simulink model "UPS_CRM_PFC"  (R2023b)
settings: Solver=FixedStepAuto  StartTime=0.0  StopTime=0.5  RelTol=1e-3
libraries: spsSeriesRLCBranchLib x7, spsVoltageMeasurementLib x5, spsUniversalBridgeLib x3, spsCurrentMeasurementLib x2, spsACVoltageSourceLib x1, simulink_extras x1, spsMeanLib x1, spsMutualInductanceLib x1, slpidlib x1, powerlib_extras x1, spsTHDLib x1, spspowerguiLib x1
settings Model: SimulationMode=accelerator  Creator=abc6820292  LastModifiedBy=Qu
settings SolverCC: ZeroCrossAlgorithm=Adaptive
settings DebuggingCC: IgnoredZcDiagnostic=none  UnconnectedInputMsg=warning  UnconnectedOutputMsg=warning  UnconnectedLineMsg=warning
settings ModelReferenceCC: EnableRefExpFcnMdlSchedulingChecks=on
settings RTWCC: DLArmComputeVersion=19.05

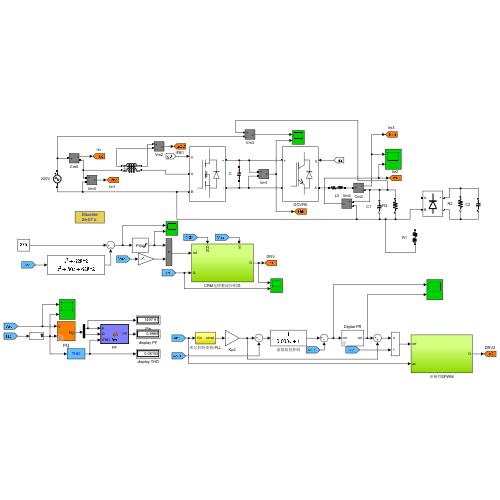
[thumbnail: Simulink's stored preview of the top-level diagram]
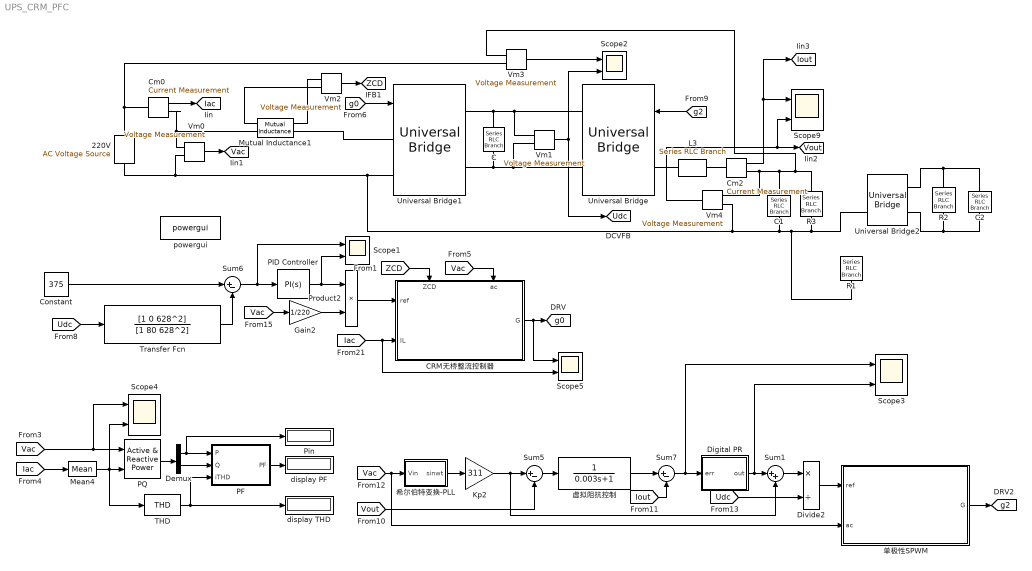
== system UPS_CRM_PFC ==
  220V : spsACVoltageSourceLib/AC Voltage Source  Amplitude=220*1.414  Phase=0  Frequency=50  SampleTime=0  Measurements=None  BusType=swing  Pref=10e3  Qref=0  Qmin=-inf  Qmax=+inf
  C : spsSeriesRLCBranchLib/Series RLC Branch  LConnTagsString=__new0  RConnTagsString=__new0  BranchType=C  Resistance=0  Inductance=0  SetiL0=off  InitialCurrent=0  Capacitance=1e-3  Setx0=on  InitialVoltage=311  Measurements=None
  C1 : spsSeriesRLCBranchLib/Series RLC Branch  LConnTagsString=__new0  RConnTagsString=__new0  BranchType=C  Resistance=1  Inductance=7e-4  SetiL0=off  InitialCurrent=0  Capacitance=8e-6  Setx0=off  InitialVoltage=0  Measurements=None
  C2 : spsSeriesRLCBranchLib/Series RLC Branch  LConnTagsString=__new0  RConnTagsString=__new0  BranchType=C  Resistance=1  Inductance=7e-4  SetiL0=off  InitialCurrent=0  Capacitance=3e-4  Setx0=on  InitialVoltage=310  Measurements=None
  CRM无桥整流控制器 : Subsystem
      settings: PortSchema="{\"entries\":[{\"content\":{\"sides\":[{\"content\":{\"connectorIds\":[\"In1\",\"In2\"]},\"type\":\"ConnectorPlacement.EquallySpacedRectSide\",\"uuid\":\"1bd7ac54-a56f-4e4b-97da-9efa063811af\"},{\"content\":{\"connectorIds\":[\"Out1\"],\"side\":\"RIGHT\"},\"type\":\"ConnectorPlacement.EquallySpacedRectSide\",\"uuid\":\"8c660721-b9a4-452b-be35-8f715241932e\"},{\"content\":{\"connectorIds\":[\"In3\",\"In4\"],\"side\":\"TOP\"},\"type\":\"ConnectorPlacement.EquallySpacedRectSide\",\"uuid\":\"028ceefa-bc2a-4c38-bf2f-a5d47b948d29\"}]},\"type\":\"ConnectorPlacement.EquallySpacedConnector\",\"uuid\":\"13f5ffb4-129e-4bc5-9f57-2ec10c2e64e6\"}],\"packageUris\":[\"http://schema.mathworks.com/mf0/Connector/R2020b\"],\"version\":\"1.0\"}"
  Cm0 : spsCurrentMeasurementLib/Current Measurement  PhasorSimulation=off  OutputType=Complex  PSBequivalent=0
  Cm2 : spsCurrentMeasurementLib/Current Measurement  PhasorSimulation=off  OutputType=Complex  PSBequivalent=0
  Constant : Constant  Value=375
  Demux : Demux  Outputs=2
  Digital PR : Subsystem  mask{Kp=8, Kr=50, Wc=5, Ts=1/20000, Upper=400, Lower=-400}
      mask DialogControl ParameterGroupVar Prompt: 参数
  Divide2 : Product  Inputs=*/
  Gain2 : Gain  Gain=1/220
  Kp2 : Gain  Gain=311
  L3 : spsSeriesRLCBranchLib/Series RLC Branch  LConnTagsString=__new0  RConnTagsString=__new0  BranchType=RL  Resistance=0.1  Inductance=1e-3  SetiL0=off  InitialCurrent=0  Capacitance=inf  Setx0=off  InitialVoltage=0  Measurements=None
  Mean4 : spsMeanLib/Mean  Freq=5000  Vinit=0  Ts=0
  Mutual Inductance1 : spsMutualInductanceLib/Mutual Inductance  LConnTagsString=a|b  RConnTagsString=A|B  TypeOfMutual=Two or three windings with equal mutual terms  NumberOfWindings=3  SelfImpedance1=[0.01 1e-4]  SelfImpedance2=[0.01 2e-4]  ThreeWindings=off  SelfImpedance3=[ 1.1 1.1e-03]  MutualImpedance=[0.05 0.99e-4]  InductanceMatrix="[1.0 0.9  0.9 ;  0.9 1.0  0.9;  0.9 0.9 1.0 ] * 1e-3"  ResistanceMatrix="[1.0 0.9  0.9 ;  0.9 1.0  0.9;  0.9 0.9 1.0 ]"  Measurements=None
  PF : MATLAB Function  TreatAsAtomicUnit=on
  PID Controller : slpidlib/PID Controller  Controller=PI  Form=Parallel  TimeDomain=Continuous-time  UseExternalTs=off  SampleTime=-1  IntegratorMethod=Forward Euler  FilterMethod=Forward Euler  ControllerParametersSource=internal  P=0.2  I=6  UseKiTs=off  D=0.005  N=100  UseFilter=on  TunerSelectOption=Transfer Function Based (PID Tuner App)  InitialConditionSource=internal  InitialConditionForIntegrator=0  InitialConditionForFilter=0  DifferentiatorICPrevScaledInput=0  ExternalReset=none  TrackingMode=off  Kt=1  LimitOutput=on  SatLimitsSource=internal  UpperSaturationLimit=200  LowerSaturationLimit=0  LinearizeAsGain=on  AntiWindupMode=clamping  Kb=1  LimitIntegrator=off  UpperIntegratorSaturationLimit=inf  LowerIntegratorSaturationLimit=-inf  POutMin=[]  POutMax=[]  IOutMin=[]  IOutMax=[]  DOutMin=[]  DOutMax=[]  NOutMin=[]  NOutMax=[]  SumOutMin=[]  SumOutMax=[]  SaturationOutMin=[]  SaturationOutMax=[]  PParamMin=[]  PParamMax=[]  IParamMin=[]  IParamMax=[]  DParamMin=[]  DParamMax=[]  NParamMin=[]  NParamMax=[]  KbParamMin=[]  KbParamMax=[]  KtParamMin=[]  KtParamMax=[]  KbOutMin=[]  KbOutMax=[]  KtOutMin=[]  KtOutMax=[]  IntegratorOutMin=[]  IntegratorOutMax=[]  FilterOutMin=[]  FilterOutMax=[]  SumI1OutMin=[]  SumI1OutMax=[]  SumI2OutMin=[]  SumI2OutMax=[]  SumI3OutMin=[]  SumI3OutMax=[]  SumI4OutMin=[]  SumI4OutMax=[]  SumDOutMin=[]  SumDOutMax=[]  DifferentiatorOutMin=[]  DifferentiatorOutMax=[]  FilterDiffOutCoefMin=[]  FilterDiffOutCoefMax=[]  ReciprocalOutMin=[]  ReciprocalOutMax=[]  SumDenOutMin=[]  SumDenOutMax=[]  SumNumOutMin=[]  SumNumOutMax=[]  DivideOutMin=[]  DivideOutMax=[]  UdiffTsProdOutMin=[]  UdiffTsProdOutMax=[]  NTsProdOutMin=[]  NTsProdOutMax=[]  UintegralTsProdOutMin=[]  UintegralTsProdOutMax=[]  UngainTsProdOutMin=[]  UngainTsProdOutMax=[]  ClampingZeroOutDataTypeStr=Inherit: Inherit via back propagation  ClampingZeroOutMin=[]  ClampingZeroOutMax=[]  FilterDenConstantOutDataTypeStr=Inherit: Inherit via back propagation  FilterDenConstantOutMin=[]  FilterDenConstantOutMax=[]  PCopyOutDataTypeStr=Inherit: Inherit via back propagation  PCopyOutMin=[]  PCopyOutMax=[]  NCopyOutDataTypeStr=Inherit: Inherit via back propagation  NCopyOutMin=[]  NCopyOutMax=[]  IntegratorContinuousStateAttributes=''  IntegratorStateMustResolveToSignalObject=off  IntegratorRTWStateStorageClass=Auto  FilterContinuousStateAttributes=''  FilterStateMustResolveToSignalObject=off  FilterRTWStateStorageClass=Auto  ParallelPVariant=InternalParameters  IdealPVariant=Disabled  IVariant=InternalParameters  DVariant=Disabled  IntegratorVariant=Continuous  SatVariant=Enabled  AWVariant=ContClampingParallel  PCopyVariant=Disabled  TRVariant=Disabled  FdbkBlocksVariant=Forward  IdealPFdbkVariant=Disabled  SatFdbkVariant=Disabled  DerivativeFilterVariant=Disabled  NVariant=Disabled  NCopyVariant=Disabled_SignalSpec  FilterICVariant=Disabled  IntegratorICVariant=InternalICs  ExternalResetVariant=Disabled  TRSumVariant=Passthrough  SumFdbkVariant=Disabled  SumVariant=Sum_PI  TsampFilterVariant=InternalTs  TsampNgainVariant=Passthrough  TsampIntegralVariant=Disabled_SignalSpec  ExternalSaturationOutDataTypeStr=Inherit: Same as second input
  PQ : powerlib_extras/Measurements/Active & Reactive Power  f1=50
  Pin : Display
      settings: Format=bank
  Product2 : Product  RndMeth=Zero
  R1 : spsSeriesRLCBranchLib/Series RLC Branch  LConnTagsString=__new0  RConnTagsString=__new0  BranchType=RL  Resistance=5  Inductance=0.04  SetiL0=off  InitialCurrent=0  Capacitance=1e-3  Setx0=off  InitialVoltage=0  Measurements=None
  R2 : spsSeriesRLCBranchLib/Series RLC Branch  LConnTagsString=__new0  RConnTagsString=__new0  BranchType=R  Resistance=50  Inductance=7e-4  SetiL0=off  InitialCurrent=0  Capacitance=1e-3  Setx0=off  InitialVoltage=0  Measurements=None
  R3 : spsSeriesRLCBranchLib/Series RLC Branch  LConnTagsString=__new0  RConnTagsString=__new0  BranchType=R  Resistance=50  Inductance=0.04  SetiL0=off  InitialCurrent=0  Capacitance=1e-3  Setx0=off  InitialVoltage=0  Measurements=None
  Scope{1..5,9} (6 alike) : Scope  NumInputPorts=2
  Sum1 : Sum  Inputs=|++
  Sum5 : Sum  Inputs=|+-
  Sum6 : Sum  Inputs=|+-
  Sum7 : Sum  Inputs=|+-
  THD : spsTHDLib/THD  Freq=50  Ts=0
  Transfer Fcn : TransferFcn  Numerator=[1 0 628^2]  Denominator=[1 80 628^2]
  Universal Bridge : spsUniversalBridgeLib/Universal Bridge  Arms=1  SnubberResistance=1e5  SnubberCapacitance=inf  Device=IGBT / Diodes  Ron=1e-3  Lon=0  ForwardVoltages="[  1  1  ]"  ForwardVoltage=0  GTOparameters=[ 10e-6 , 20e-6 ]  IGBTparameters=[ 1e-6 , 2e-6 ]  Measurements=None  Measurements_2=None  converterType=Rectifier
  Universal Bridge1 : spsUniversalBridgeLib/Universal Bridge  Arms=2  SnubberResistance=1e5  SnubberCapacitance=inf  Device=MOSFET / Diodes  Ron=1e-3  Lon=0  ForwardVoltages="[  1  1  ]"  ForwardVoltage=0  GTOparameters=[ 10e-6 , 20e-6 ]  IGBTparameters=[ 1e-6 , 2e-6 ]  Measurements=None  Measurements_2=None  converterType=Rectifier
  Universal Bridge2 : spsUniversalBridgeLib/Universal Bridge  Arms=2  SnubberResistance=1e5  SnubberCapacitance=inf  Device=Diodes  Ron=1e-3  Lon=0  ForwardVoltages="[  1  1  ]"  ForwardVoltage=1  GTOparameters=[ 10e-6 , 20e-6 ]  IGBTparameters=[ 1e-6 , 2e-6 ]  Measurements=None  Measurements_2=None  converterType=Rectifier
  Vm{0..4} (5 alike) : spsVoltageMeasurementLib/Voltage Measurement  PhasorSimulation=off  OutputType=Complex  PSBequivalent=0
  display PF : Display
  display THD : Display
  powergui : spspowerguiLib/powergui  SimulationMode=Discrete  SampleTime=2e-7  frequency=60  Iterations=50  frequencyindice=0  Pbase=100e6  ErrMax=1e-4  UnitsV=kV  UnitsW=MW  buscounter=0  FunctionMessages=off  echomessages=off  EnableUseOfTLC=off  CurrentSourceSwitches=off  DisableSnubberDevices=off  DisableRonSwitches=off  DisableVfSwitches=off  DisplayEquations=off  AutomaticDiscreteSolvers=off  SolverType=Tustin/Backward Euler (TBE)  Interpol=off  ExternalGateDelay=off  methode=off  Ts=0  x0status=blocks  SPID=off  SwTol=0  HookPort=off  NonlinearTolerance=1e-4  nMaxIteration=100  ContinueOnMaxIteration=off  RestoreLinks=warning  ResistiveCurrentMeasurement=off  Frange=[0:2:500]  Ylog=off  Xlog=on  ShowGrid=off  save=off  variable=ZData  structure=QQQQQ  ZoomFFT=off  StartTime=0.5  cycles=15  DisplayStyle=1  fundamental=50  FreqAxis=off  MaxFrequency=1000  frequencyindicesteady=1  RmsSteady=1  display=off
  单极性SPWM : Subsystem
  希尔伯特变换-PLL : Subsystem
  虚拟阻抗控制 : TransferFcn  Numerator=1  Denominator=[0.003 1]
  tag scope: Iac=global, Iout=global, Udc=global, Vac=global, Vout=global, ZCD=global, g0=global, g2=global
  wires:
  Transfer Fcn/1 -> Sum6/2
  PF/1(PF) -> display PF/1
  [Iac] -> Mean4/1
  Gain2/1 -> Product2/2
  Demux/1 -> Pin/1, PF/1(P)
  Constant/1 -> Sum6/1
  [Vac] -> Scope4/1, PQ/1
  PID Controller/1 -> Scope1/2, Product2/1
  Sum6/1 -> PID Controller/1, Scope1/1
  Vm0/1 -> [Vac]
  Mean4/1 -> THD/1, Scope4/2, PQ/2
  Cm0/1 -> [Iac]
  PQ/1 -> Demux/1
  Demux/2 -> PF/2(Q)
  THD/1 -> display THD/1, PF/3(iTHD)
  Vm1/1 -> [Udc], Scope2/2
  [Udc] -> Transfer Fcn/1
  Cm2/1 -> [Iout], Scope9/1
  [Vout] -> Sum5/2
  [Iout] -> Sum7/2
  Vm4/1 -> [Vout], Scope9/2
  [Vac] -> 单极性SPWM/2(ac), 希尔伯特变换-PLL/1(Vin)
  Sum5/1 -> 虚拟阻抗控制/1
  [Udc] -> Divide2/2
  Vm2/1 -> [ZCD]
  [Iac] -> CRM无桥整流控制器/2(IL), Scope5/2
  Product2/1 -> CRM无桥整流控制器/1(ref)
  CRM无桥整流控制器/1(G) -> Scope5/1, [g0]
  [ZCD] -> CRM无桥整流控制器/3(ZCD)
  [Vac] -> Gain2/1
  Vm3/1 -> Scope2/1
  [g0] -> Universal Bridge1/1
  [Vac] -> CRM无桥整流控制器/4(ac)
  [g2] -> Universal Bridge/1
  单极性SPWM/1(G) -> [g2]
  Sum7/1 -> Digital PR/1(err), Scope3/1
  Digital PR/1(out) -> Scope3/2, Sum1/1
  Sum1/1 -> Divide2/1
  Kp2/1 -> Sum5/1, Sum1/2
  Divide2/1 -> 单极性SPWM/1(ref)
  希尔伯特变换-PLL/1(sinwt) -> Kp2/1
  虚拟阻抗控制/1 -> Sum7/1
  connections:
  Cm0/RConn1 -- Vm0/LConn1 -- Mutual Inductance1/LConn2
  C1/RConn1 -- R3/RConn1 -- Universal Bridge2/LConn2 -- R1/RConn1 -- Universal Bridge1/LConn2 -- 220V/LConn1 -- Vm0/LConn2 -- Vm4/LConn2
  Vm1/LConn1 -- Universal Bridge/RConn1 -- Universal Bridge1/RConn1 -- C/LConn1
  L3/LConn1 -- Universal Bridge/LConn1
  Cm2/LConn1 -- L3/RConn1
  Cm2/RConn1 -- R3/LConn1 -- Vm3/LConn1 -- C1/LConn1 -- Vm4/LConn1
  Cm0/LConn1 -- 220V/RConn1 -- Vm3/LConn2
  Vm1/LConn2 -- Universal Bridge/RConn2 -- Universal Bridge1/RConn2 -- C/RConn1
  Mutual Inductance1/RConn1 -- Vm2/LConn1
  Vm2/LConn2 -- Mutual Inductance1/LConn1
  Mutual Inductance1/RConn2 -- Universal Bridge1/LConn1
  R2/LConn1 -- Universal Bridge2/RConn1 -- C2/LConn1
  R2/RConn1 -- Universal Bridge2/RConn2 -- C2/RConn1

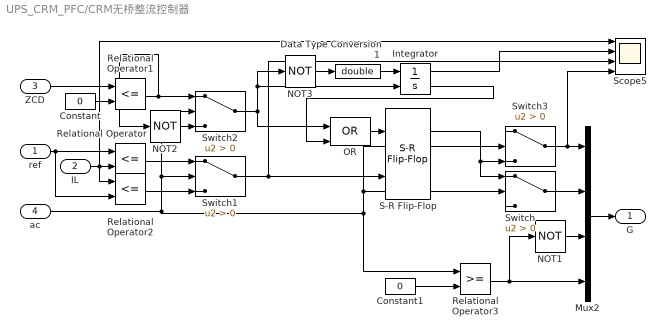
== system UPS_CRM_PFC/CRM无桥整流控制器 ==
  ref : Inport
  IL : Inport  Port=2
  ZCD : Inport  Port=3
  ac : Inport  Port=4
  Constant : Constant  Value=0
  Constant1 : Constant  Value=0
  Data Type Conversion1 : DataTypeConversion  OutDataTypeStr=double  SaturateOnIntegerOverflow=off  RndMeth=Floor
  Integrator : Integrator  ExternalReset=rising  LimitOutput=on  UpperSaturationLimit=1e-4  ShowSaturationPort=on
  Mux2 : Mux
  NOT1 : Logic  Operator=NOT  IconShape=distinctive  AllPortsSameDT=off  OutDataTypeStr=boolean
  NOT2 : Logic  Operator=NOT  IconShape=distinctive  AllPortsSameDT=off  OutDataTypeStr=boolean
  NOT3 : Logic  Operator=NOT  IconShape=distinctive  AllPortsSameDT=off  OutDataTypeStr=boolean
  OR : Logic  Operator=OR  IconShape=distinctive  AllPortsSameDT=off  OutDataTypeStr=boolean
  Relational Operator : RelationalOperator  Operator=<=  OutDataTypeStr=boolean  InputSameDT=off
  Relational Operator1 : RelationalOperator  Operator=<=  OutDataTypeStr=boolean  InputSameDT=off
  Relational Operator2 : RelationalOperator  Operator=<=  OutDataTypeStr=boolean  InputSameDT=off
  Relational Operator3 : RelationalOperator  OutDataTypeStr=boolean  InputSameDT=off
  S-R Flip-Flop : simulink_extras/Flip Flops/S-R Flip-Flop  initial_condition=0
  Scope5 : Scope  NumInputPorts=4
  Switch{,1..3} (4 alike) : Switch  Criteria=u2 > Threshold  SaturateOnIntegerOverflow=off  InputSameDT=off
  G : Outport
  wires:
  NOT2/1 -> Switch2/3
  Switch3/1 -> Scope5/4, Mux2/1
  Switch/1 -> Mux2/2
  S-R Flip-Flop/1 -> Switch/1, Switch3/3
  Relational Operator1/1 -> Switch2/1, NOT2/1
  ZCD/1 -> Relational Operator1/1
  Relational Operator2/1 -> Switch1/3
  Switch1/1 -> Scope5/3, S-R Flip-Flop/2
  Relational Operator/1 -> Switch1/1
  Relational Operator3/1 -> Mux2/4, NOT1/1
  Constant1/1 -> Relational Operator3/2
  Mux2/1 -> G/1
  ac/1 -> Switch1/2, Switch2/2, Switch/2, Switch3/2, Relational Operator3/1
  Constant/1 -> Relational Operator1/2
  IL/1 -> Relational Operator2/1, Scope5/1, Relational Operator/2
  ref/1 -> Relational Operator/1, Relational Operator2/2
  NOT1/1 -> Mux2/3
  OR/1 -> S-R Flip-Flop/1
  Switch2/1 -> Integrator/2, NOT3/1, OR/1
  Integrator/1 -> Scope5/2
  Integrator/2 -> OR/2
  NOT3/1 -> Data Type Conversion1/1
  Data Type Conversion1/1 -> Integrator/1

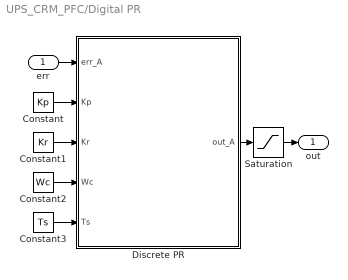
== system UPS_CRM_PFC/Digital PR ==
  err : Inport
  Constant : Constant  Value=Kp
  Constant1 : Constant  Value=Kr
  Constant2 : Constant  Value=Wc
  Constant3 : Constant  Value=Ts
  Discrete PR : MATLAB Function  TreatAsAtomicUnit=on
  Saturation : Saturate  UpperLimit=Upper  LowerLimit=Lower
  out : Outport
  wires:
  Constant1/1 -> Discrete PR/3(Kr)
  Constant3/1 -> Discrete PR/5(Ts)
  Constant/1 -> Discrete PR/2(Kp)
  Constant2/1 -> Discrete PR/4(Wc)
  Discrete PR/1(out_A) -> Saturation/1
  Saturation/1 -> out/1
  err/1 -> Discrete PR/1(err_A)

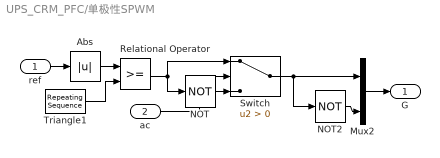
== system UPS_CRM_PFC/单极性SPWM ==
  ref : Inport
  ac : Inport  Port=2
  Abs : Abs  SaturateOnIntegerOverflow=off
  Mux2 : Mux  Inputs=2
  NOT : Logic  Operator=NOT  IconShape=distinctive  AllPortsSameDT=off  OutDataTypeStr=boolean
  NOT2 : Logic  Operator=NOT  IconShape=distinctive  AllPortsSameDT=off  OutDataTypeStr=boolean
  Relational Operator : RelationalOperator  OutDataTypeStr=boolean  InputSameDT=off
  Switch : Switch  Criteria=u2 > Threshold  SaturateOnIntegerOverflow=off  InputSameDT=off
  Triangle1 : simulink/Sources/Repeating Sequence  rep_seq_t=[0 1/20000/2 1/20000]  rep_seq_y=[0 1 0]
  G : Outport
  wires:
  Triangle1/1 -> Relational Operator/2
  Mux2/1 -> G/1
  Relational Operator/1 -> Switch/1, NOT/1
  Abs/1 -> Relational Operator/1
  NOT/1 -> Switch/3
  ref/1 -> Abs/1
  ac/1 -> Switch/2
  Switch/1 -> NOT2/1, Mux2/1
  NOT2/1 -> Mux2/2

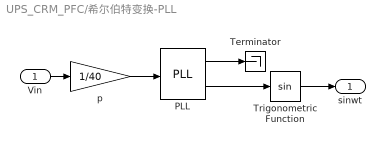
== system UPS_CRM_PFC/希尔伯特变换-PLL ==
  Vin : Inport
  PLL : spsPLLLib/PLL  Fmin=45  Par_Init=[0, 50]  ParK=[180, 3200, 1]  TcD=1e-4  MaxRateChangeFreq=12  FilterCutOffFreq=25  Ts=0  AGC=on
  Terminator : Terminator
  Trigonometric Function : Trigonometry
  p : Gain  Gain=1/40
  sinwt : Outport
  wires:
  PLL/2 -> Trigonometric Function/1
  PLL/1 -> Terminator/1
  p/1 -> PLL/1
  Trigonometric Function/1 -> sinwt/1
  Vin/1 -> p/1

== matlab function UPS_CRM_PFC/PF ==
  data: P input; PF output; Q input; iTHD input
function PF = fcn(P,Q,iTHD)
% This block supports an embeddable subset of the MATLAB language.
% See the help menu for details. 
PF=(P/sqrt(P*P+Q*Q))/(sqrt(1+iTHD*iTHD));

== matlab function UPS_CRM_PFC/Digital PR/Discrete PR ==
  settings: updateMethod=DISCRETE  sampleTime=Ts
  data: err_A input; out_A output; Kp input; Kr input; Wc input; Ts input
function out_A  = fcn(err_A, Kp, Kr, Wc, Ts)

W0 = 50*2*pi;


persistent err_A1;
persistent err_A2;
persistent out_A1;
persistent out_A2;


%%对三相静态变量初始化
if isempty(err_A1)
    err_A1 = 0;
end
if isempty(err_A2)
    err_A2 = 0;
end
if isempty(out_A1)
    out_A1 = 0;
end
if isempty(out_A2)
    out_A2 = 0;
end


%%Discrete
t1 = Wc * Ts;
t2 = W0^2 * Ts^2;
t3 = t2 + 4*t1 + 4;

b0 = (Kp*t2 + 4*(Kp+Kr)*t1 + 4*Kp) / t3;
b1 = (2*Kp*t2 - 8*Kp) / t3;
b2 = (Kp*t2 + 4*Kp - 4*(Kp+Kr)*t1) / t3;
a1 = (2*t2 - 8) / t3;
a2 = (t2 - 4*t1 + 4) / t3;
%%限制输出
if b0>3000
    b0=0;
end
if b0<-3000
    b0=0;
end

%%计算输出量
out_A = b0*err_A + b1*err_A1 + b2*err_A2 - a1*out_A1 - a2*out_A2;
out_A2 = out_A1;
out_A1 = out_A;
err_A2 = err_A1;
err_A1 = err_A;
